simulink library "WECSim_Lib_PTOSim"  (R2020b)
settings: Solver=ode45  StartTime=0.0  StopTime=10.0  RelTol=1e-3  EnableMultiTasking=on
undefined symbols (not defined in the file or in its folder): DiscIntNeverNeededParam, magnitude, ptoSim, simu
libraries: $bdroot x3, simulink x2
(part 1 of 2)
settings Model: RequirementInfo="{}  %GIDa_42666abb_d6d9_408c_ae24_f6520282b61c"  Creator=sor  LastModifiedBy=akeeste
settings DataIOCC: LimitDataPoints=on  SaveFormat=Array  ReturnWorkspaceOutputs=off
settings OptimizationCC: LifeSpan=inf
settings DebuggingCC: SolverPrmCheckMsg=warning  AllowSymbolicDim=off  SFUnexpectedBacktrackingDiag=warning  SFNoUnconditionalDefaultTransitionDiag=warning  SFExecutionAtInitializationDiag=none  ArithmeticOperatorsInVariantConditions=warning
settings HardwareCC: ProdBitPerPointer=32  ProdBitPerSizeT=32  ProdBitPerPtrDiffT=32  ProdLargestAtomicFloat=None  ProdIntDivRoundTo=Undefined  ProdEndianess=Unspecified  ProdWordSize=32  ProdHWDeviceType=32-bit Generic
settings ModelReferenceCC: PropagateSignalLabelsOutOfModel=off
settings SFSimCC: SimUseLocalCustomCode=off  CustomCodeUndefinedFunction=UseInterfaceOnly
settings RTWCC: RTWUseLocalCustomCode=off
settings CodeAppCC: StateflowObjectComments=on
settings GRTTargetCC: TargetLangStandard=C89/C90 (ANSI)
settings ConfigComp: CovMetricSettings=dw  CovSaveCumulativeToWorkspaceVar=on  CovSaveSingleToWorkspaceVar=on  CovExternalEMLEnable=off  CovSFcnEnable=off

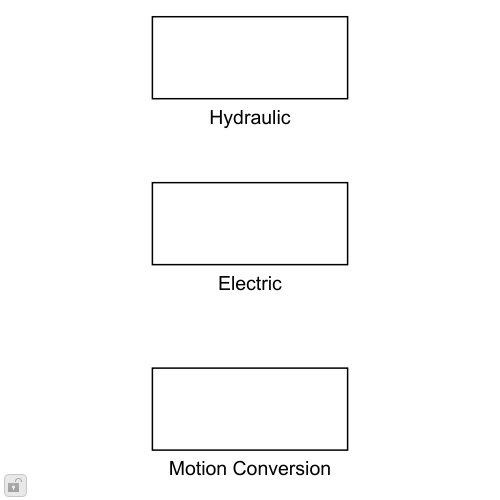
[thumbnail: Simulink's stored preview of the top-level diagram]
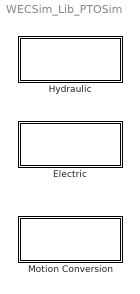
== system WECSim_Lib_PTOSim ==
  Electric : Subsystem  RequirementInfo="{}  %GIDa_5439fdb4_7c29_433c_8677_23bf92e18f11"
  Hydraulic : Subsystem  RequirementInfo={} %GIDa_f12a42eb_b9cb_4818_b573_b7dee4183a3b
  Motion Conversion : Subsystem

== system WECSim_Lib_PTOSim/Electric ==
  Direct Drive Linear Generator : Subsystem  mask{ptoSim=ptoSim(1), InputFiletext=Use WEC-Sim input file to define Direct Drive Linear Generator parameters, Rs=0, Ls=0, Rload=0, Bfric=0, tau_p=0, theta_d_0=0, lambda_sd_0=0, lambda_sq_0=0, lambda_fd=0}
      mask prompts: ptoSim "Direct Drive Linear Generator Name"; Rs "Winding resistance [ohm]"; Ls "Winding inductance [H]"; Rload "External load resistance [ohm]"; Bfric "Friction coefficient [kg/s]"; tau_p "Magnet pole pitch [m]"; theta_d_0 "Initial rotor frame angle [rad]"; lambda_sd_0 "Initial stator d-axis flow linkage"; lambda_sq_0 "Initial stator q-axis flow linkage"; lambda_fd "Flow linkage fd"
      mask init:
      | if exist('ptoSim','var')
      |     h=[gcb '/To Workspace'];
      |     responseName=['ptoSim' num2str(ptoSim.number) '_out'];
      |     set_param(h,'VariableName',responseName);
      | end
      | clear h responseName
      mask DialogControl CustomParameterGroup Prompt: Custom Parameters
      mask DialogControl LGParameters Prompt: Linear Generator Parameters
      mask Display: image('DirectDriveLinearGenerator.png'); % Use "Edit Image" on toolstrip to change.
  Direct Drive Rotary Generator : Subsystem  mask{ptoSim=ptoSim(1)}
      mask prompts: ptoSim "Direct Drive Rotary Generator Name"
      mask init:
      | if exist('ptoSim','var')
      |     h=[gcb '/To Workspace'];
      |     responseName=['ptoSim' num2str(ptoSim.number) '_out'];
      |     set_param(h,'VariableName',responseName);
      | end
      | clear h responseName
      mask Display: image('DirectDriveRotaryGenerator.png'); % Use "Edit Image" on toolstrip to change.
  Electric Generator Equivalent Circuit : Subsystem  mask{ptoSim=ptoSim(1), InputFiletext=Use WEC-Sim input file to define Electric Machine parameters, Ra=0, La=0, Ke=0, bShaft=0, Jem=0}
      mask prompts: ptoSim "Electric Machine Name"; Ra "Armature Resistance [ohm]"; La "Armature Inductance [H]"; Ke "Back-emf or Torque constant [V/(rad/s)]"; bShaft "Rotor Damping [N s/m]"; Jem "Rotor Inertia [kg m^2]"
      mask init:
      | if exist('ptoSim','var')
      |     h=[gcb '/To Workspace'];
      |     responseName=['ptoSim' num2str(ptoSim.number) '_out'];
      |     set_param(h,'VariableName',responseName);
      | end
      | clear h responseName
      settings: PortSchema="{\"entries\":[{\"content\":{\"sides\":[{\"content\":{\"connectorIds\":[\"In1\"]},\"type\":\"ConnectorPlacement.EquallySpacedRectSide\",\"uuid\":\"38b15b7d-d952-45b6-9eb0-5d473736364e\"},{\"content\":{\"connectorIds\":[\"Out1\"],\"side\":\"RIGHT\"},\"type\":\"ConnectorPlacement.EquallySpacedRectSide\",\"uuid\":\"de64adb9-f2de-4dd5-b519-c63af884483d\"},{\"content\":{\"connectorIds\":[\"In2\"],\"side\":\"TOP\"},\"type\":\"ConnectorPlacement.EquallySpacedRectSide\",\"uuid\":\"eaa9506a-5e37-41b4-975c-a8d526700d36\"},{\"content\":{\"connectorIds\":[],\"side\":\"HIDDEN\"},\"type\":\"ConnectorPlacement.EquallySpacedRectSide\",\"uuid\":\"f8da1221-e5bc-4844-b966-beaaa1d6bf60\"}]},\"type\":\"ConnectorPlacement.EquallySpacedConnector\",\"uuid\":\"4da2b473-e94d-42dc-9143-64fbcbf5d9e1\"}],\"packageUris\":[\"http://schema.mathworks.com/mf0/Connector/R2020b\"],\"version\":\"1.0\"}"
      mask DialogControl CustomParameterGroup Prompt: Custom Parameters
      mask DialogControl EMParameters Prompt: Electric Machine Parameters
      mask Display: image('ElectricMotor.png'); % Use "Edit Image" on toolstrip to change.
  Simple Direct Drive PTO : Subsystem  mask{ptoSim=ptoSim(1)}
      mask prompts: ptoSim "Simple Direct Drive PTO"
      mask init:
      | if exist('ptoSim', 'var')
      |     h=[gcb '/To Workspace'];
      |     responseName=['ptoSim' num2str(ptoSim.number) '_out'];
      |     set_param(h,'VariableName',responseName);
      | end
      | clear h responseName
      mask Display: image('simpleDDPTO.png'); % Use "Edit Image" on toolstrip to change.

== system WECSim_Lib_PTOSim/Hydraulic ==
  Check Valve : Subsystem  mask{ptoSim=ptoSim(1)}
      mask prompts: ptoSim "Chack Valve Name"
      mask init:
      | if exist('ptoSim','var')
      |     h=[gcb '/To Workspace'];
      |     responseName=['ptoSim' num2str(ptoSim.number) '_out'];
      |     set_param(h,'VariableName',responseName);
      | end
      | clear h responseName
      mask Display: image('CheckValve.png'); % Use "Edit Image" on toolstrip to change.
  Compressible Fluid Piston : Subsystem  mask{ptoSim=ptoSim(1)}
      mask prompts: ptoSim "Piston Name"
      mask help:
      | PTO-Sim Compressible Fluid Piston
      |
      | This block simualtes a hydraulic cylinder using a compressible fluid model. The block inputs are Response, QA and QB. Response is the signal output of the block Rotational PTO Actuation Force. QA and QB are the flow rate for port A and port B of the cylinder. The outputs of the block are ForcePTO, PA, and PB.
      mask init:
      | if exist('ptoSim','var')
      |     h=[gcb '/To Workspace'];
      |     responseName=['ptoSim' num2str(ptoSim.number) '_out'];
      |     set_param(h,'VariableName',responseName);
      | end
      | clear h responseName
      settings: PortSchema="{\"entries\":[{\"content\":{\"sides\":[{\"content\":{\"connectorIds\":[\"In1\",\"In2\"]},\"type\":\"ConnectorPlacement.EquallySpacedRectSide\",\"uuid\":\"572dbc7c-8f4c-46fc-9000-663c89355fbd\"},{\"content\":{\"connectorIds\":[\"Out1\",\"Out2\",\"Out3\"],\"side\":\"RIGHT\"},\"type\":\"ConnectorPlacement.EquallySpacedRectSide\",\"uuid\":\"3b7821ce-a540-4de1-8f34-0d55375c774c\"},{\"content\":{\"connectorIds\":[\"In3\"],\"side\":\"TOP\"},\"type\":\"ConnectorPlacement.EquallySpacedRectSide\",\"uuid\":\"b6f5c275-868d-447d-b609-cdda14e9f222\"},{\"content\":{\"connectorIds\":[],\"side\":\"HIDDEN\"},\"type\":\"ConnectorPlacement.EquallySpacedRectSide\",\"uuid\":\"5b34aa5d-01fb-4d75-9f22-3e4ce64ee132\"}]},\"type\":\"ConnectorPlacement.EquallySpacedConnector\",\"uuid\":\"5b16a2f7-6624-4a26-89bf-8d87cef610e1\"}],\"packageUris\":[\"http://schema.mathworks.com/mf0/Connector/R2020b\"],\"version\":\"1.0\"}"
      mask Help:
      | This block simualtes a hydraulic cylinder using a compressible fluid model. The block inputs are Response and HydraulicInput. Response is the signal output of the block Rotational PTO Actuation Force. HydraulicInput is a two signal vector with the information of the flow rate for port A and port B of the cylinder. The output of the block is ptoSimOutput, which is a three signal vector with pressureA, pressureB, and forcePTO.
      | 
      | The outputs are calculated using the model presented in the following link: http://wec-sim.github.io/WEC-Sim/master/user/advanced_features.html#pto-sim
      mask Display: image('DoubleActingPiston.png'); % Use "Edit Image" on toolstrip to change.
  Gas-Charged Hydraulic Accumulator : Subsystem  mask{ptoSim=ptoSim(1)}
      mask prompts: ptoSim "Accumulator Name"
      mask init:
      | if exist('ptoSim','var')
      |     h=[gcb '/To Workspace'];
      |     responseName=['ptoSim' num2str(ptoSim.number) '_out'];
      |     set_param(h,'VariableName',responseName);
      | end
      | clear h responseName
      mask Display: image('GasAccumulator.png'); % Use "Edit Image" on toolstrip to change.
  Hydraulic Motor : Subsystem  Variant=on  AllowZeroVariantControls=on  mask{ptoSim=ptoSim(1)}
      mask prompts: ptoSim "Hydraulic Motor Name"
      mask init:
      | if exist('ptoSim','var')
      |     %%
      |     % Analytical efficiency
      |     %%
      |     h = [gcb '/AnalyticalEfficiencyModel'];
      |     responseName = ['sv_b' num2str(ptoSim.number) '_AnalyticalEfficiency'];
      |     set_param(h,'VariantControl',responseName);
      |     %%
      |     % Tabulated Efficiency
      |     %%
      |     h = [gcb '/TabulatedEfficiency'];
      |     responseName = ['sv_b' num2str(ptoSim.number) '_TabulatedEfficiency'];
      |     set_param(h,'VariantControl',responseName);
      |     %%
      |     % Set zero active variant controls to prevent label issue (works 2017b+)
      |     %%
      |     set_param(gcb,'AllowZeroVariantControls','on');
      |     %%
      |     h=[gcb '/TabulatedEfficiency/To Workspace'];
      |     responseName=['ptoSim' num2str(ptoSim.number) '_out'];
      |     set_param(h,'VariableName',responseName);
      |     %%
      |     h=[gcb '/AnalyticalEfficiencyModel/To Workspace'];
      |     responseName=['ptoSim' num2str(ptoSim.number) '_out'];
      |     set_param(h,'VariableName',responseName);
      | end
      | clear h responseName
      mask Display: image('VariableDisplacementHydraulicMotor.png'); % Use "Edit Image" on toolstrip to change.
  Rectifying Check Valve : Subsystem  mask{ptoSim=ptoSim(1)}
      mask prompts: ptoSim "Rectifying Valve Name"
      mask init:
      | if exist('ptoSim','var')
      |     h=[gcb '/To Workspace'];
      |     responseName=['ptoSim' num2str(ptoSim.number) '_out'];
      |     set_param(h,'VariableName',responseName);
      | end
      | clear h responseName
      mask Display: image('RectifyingCheckValve.png'); % Use "Edit Image" on toolstrip to change.

== system WECSim_Lib_PTOSim/Motion Conversion ==
  Rotary to Linear Adjustable Rod : Subsystem  mask{ptoSim=ptoSim(1)}
      mask prompts: ptoSim "Adjustable Rod Name"
      mask init:
      | if exist('ptoSim','var')
      |     h=[gcb '/To Workspace'];
      |     responseName=['ptoSim' num2str(ptoSim.number) '_out'];
      |     set_param(h,'VariableName',responseName);
      | end
      | clear h responseName
  Rotary to Linear Crank : Subsystem  mask{ptoSim=ptoSim(1)}
      mask prompts: ptoSim "Linear Crank Name"
      mask init:
      | if exist('ptoSim','var')
      |     h=[gcb '/To Workspace'];
      |     responseName=['ptoSim' num2str(ptoSim.number) '_out'];
      |     set_param(h,'VariableName',responseName);
      | end
      | clear h responseName

== system WECSim_Lib_PTOSim/Electric/Direct Drive Linear Generator ==
  Response : Inport
  ABCtoDQ : Subsystem
  ABCtoDQ2 : Subsystem
  Add : Sum
  Bus Creator : BusCreator  Inputs=11
  Bus Selector : BusSelector  OutputSignals=velocity
  Demux : Demux  Outputs=3
  Demux1 : Demux  Outputs=3
  Gain : Gain  Gain=-1
  Gain5 : Gain  Gain=2*pi/(2*ptoSim.directLinearGenerator.tau_p)
  Integrator2 : Integrator  InitialCondition=ptoSim.directLinearGenerator.theta_d_0
  Losses : Subsystem
  Product : Product
  Selector1 : Selector  InputPortWidth=6  IndexOptions=Index vector (dialog)  Indices=3  OutputSizes=1
  Subsystem : Subsystem
  Subsystem1 : Subsystem
  Terminator : Terminator
  To Workspace : ToWorkspace  VariableName=ptoSim1_out  SaveFormat=Structure With Time  SampleTime=simu.dtOut
  Force : Outport
  wires:
  Bus Selector/1 -> Selector1/1  "<velocity>"
  Response/1 -> Bus Selector/1
  Gain5/1 -> Subsystem/2(wd), Integrator2/1  "wsyn"
  Selector1/1 -> Bus Creator/10, Product/1, Losses/1(vel), Gain5/1  "vel"
  Integrator2/1 -> ABCtoDQ/1(theta_d), ABCtoDQ2/1(theta_d)
  ABCtoDQ/1(DQ) -> Subsystem/1(vsdq)
  Losses/1(fricForce) -> Add/1, Bus Creator/3  "fricForce"
  Subsystem/1(Fem) -> Add/2
  Subsystem/2(isdq) -> ABCtoDQ2/2(dq)
  ABCtoDQ2/1(abc) -> Demux/1, Subsystem1/1(Iabc)
  Subsystem1/1(Vabc) -> Demux1/1, ABCtoDQ/2(ABC)
  Add/1 -> Product/2, Force/1, Bus Creator/2  "force"
  Product/1 -> Gain/1
  Gain/1 -> Terminator/1, Bus Creator/1  "absPower"
  Bus Creator/1 -> To Workspace/1
  Demux/1 -> Bus Creator/4  "Ia"
  Demux/2 -> Bus Creator/5  "Ib"
  Demux/3 -> Bus Creator/6  "Ic"
  Demux1/3 -> Bus Creator/9  "Vc"
  Demux1/2 -> Bus Creator/8  "Vb"
  Demux1/1 -> Bus Creator/7  "Va"
  Subsystem1/2(elecPower) -> Bus Creator/11  "elecPower"

== system WECSim_Lib_PTOSim/Electric/Direct Drive Rotary Generator ==
  Response : Inport
  ABCtoDQ : Subsystem  AncestorBlock=PTOSim_Lib/Electric/Direct Drive Linear Generator/ABCtoDQ
  ABCtoDQ2 : Subsystem  AncestorBlock=PTOSim_Lib/Electric/Direct Drive Linear Generator/ABCtoDQ2
  Add : Sum
  Bus Creator : BusCreator  Inputs=11
  Bus Selector : BusSelector  OutputSignals=velocity
  Demux : Demux  Outputs=3
  Demux1 : Demux  Outputs=3
  Gain : Gain  Gain=-1
  Gain5 : Gain  Gain=2*pi*ptoSim.directRotaryGenerator.radius/(2*ptoSim.directRotaryGenerator.tau_p)
  Integrator2 : Integrator  InitialCondition=ptoSim.directRotaryGenerator.theta_d_0
  Losses : Subsystem  AncestorBlock=PTOSim_Lib/Electric/Direct Drive Linear Generator/Losses
  Product : Product
  Selector1 : Selector  InputPortWidth=6  IndexOptions=Index vector (dialog)  Indices=3  OutputSizes=1
  Subsystem : Subsystem  AncestorBlock=PTOSim_Lib/Electric/Direct Drive Linear Generator/Subsystem
  Subsystem1 : Subsystem  AncestorBlock=PTOSim_Lib/Electric/Direct Drive Linear Generator/Subsystem1
  Terminator : Terminator
  To Workspace : ToWorkspace  VariableName=ptoSim1_out  SaveFormat=Structure With Time  SampleTime=simu.dtOut
  Torque : Outport
  wires:
  Demux1/2 -> Bus Creator/8  "Vb"
  Selector1/1 -> Bus Creator/10, Product/1, Losses/1(vel), Gain5/1  "vel"
  Subsystem/1(Fem) -> Add/2
  Integrator2/1 -> ABCtoDQ/1(theta_d), ABCtoDQ2/1(theta_d)
  Subsystem/2(isdq) -> ABCtoDQ2/2(dq)
  Gain5/1 -> Subsystem/2(wd), Integrator2/1  "wsyn"
  Subsystem1/1(Vabc) -> Demux1/1, ABCtoDQ/2(ABC)
  Bus Creator/1 -> To Workspace/1
  Demux/3 -> Bus Creator/6  "Ic"
  Add/1 -> Product/2, Torque/1, Bus Creator/2  "Torque"
  Bus Selector/1 -> Selector1/1  "<velocity>"
  Losses/1(fricTorque) -> Add/1, Bus Creator/3  "fricTorque"
  Demux/1 -> Bus Creator/4  "Ia"
  Gain/1 -> Terminator/1, Bus Creator/1  "absPower"
  Demux1/3 -> Bus Creator/9  "Vc"
  Product/1 -> Gain/1
  Response/1 -> Bus Selector/1
  ABCtoDQ2/1(abc) -> Demux/1, Subsystem1/1(Iabc)
  Demux1/1 -> Bus Creator/7  "Va"
  Subsystem1/2(elecPower) -> Bus Creator/11  "elecPower"
  Demux/2 -> Bus Creator/5  "Ib"
  ABCtoDQ/1(DQ) -> Subsystem/1(vsdq)

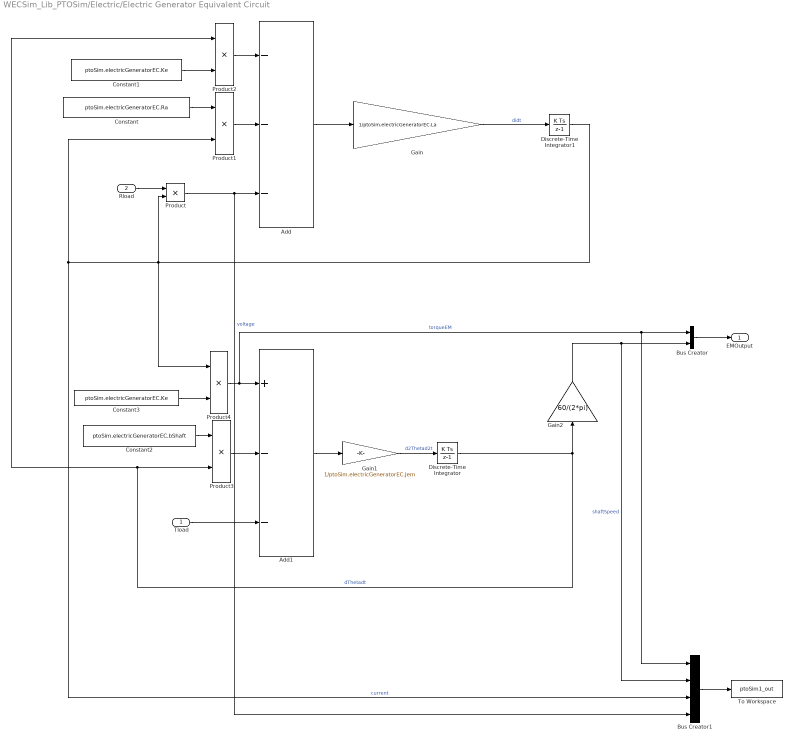
== system WECSim_Lib_PTOSim/Electric/Electric Generator Equivalent Circuit ==
  Tload : Inport
  Rload : Inport  Port=2
  Add : Sum  Inputs=---
  Add1 : Sum  Inputs=+--
  Bus Creator : BusCreator  Inputs=2
  Bus Creator1 : BusCreator  Inputs=4
  Constant : Constant  Value=ptoSim.electricGeneratorEC.Ra
  Constant1 : Constant  Value=ptoSim.electricGeneratorEC.Ke
  Constant2 : Constant  Value=ptoSim.electricGeneratorEC.bShaft
  Constant3 : Constant  Value=ptoSim.electricGeneratorEC.Ke
  Discrete-Time Integrator : DiscreteIntegrator  InitialCondition=(2*pi/60)*ptoSim.electricGeneratorEC.wShaftIni  SampleTime=-1  ICPrevOutput=DiscIntNeverNeededParam  ICPrevScaledInput=DiscIntNeverNeededParam
  Discrete-Time Integrator1 : DiscreteIntegrator  InitialCondition=ptoSim.electricGeneratorEC.currentIni  SampleTime=-1  ICPrevOutput=DiscIntNeverNeededParam  ICPrevScaledInput=DiscIntNeverNeededParam
  Gain : Gain  Gain=1/ptoSim.electricGeneratorEC.La
  Gain1 : Gain  Gain=1/ptoSim.electricGeneratorEC.Jem
  Gain2 : Gain  Gain=60/(2*pi)
  Product{,1..4} (5 alike) : Product
  To Workspace : ToWorkspace  VariableName=ptoSim1_out  SaveFormat=Structure With Time  SampleTime=simu.dtOut
  EMOutput : Outport
  wires:
  Add/1 -> Gain/1
  Gain/1 -> Discrete-Time Integrator1/1  "didt"
  Rload/1 -> Product/1
  Discrete-Time Integrator1/1 -> Product4/1, Product/2, Bus Creator1/3, Product1/2  "current"
  Product/1 -> Bus Creator1/4, Add/3  "voltage"
  Product1/1 -> Add/2
  Constant/1 -> Product1/1
  Product2/1 -> Add/1
  Constant1/1 -> Product2/2
  Tload/1 -> Add1/3
  Add1/1 -> Gain1/1
  Gain1/1 -> Discrete-Time Integrator/1  "d2Thetad2t"
  Product3/1 -> Add1/2
  Constant2/1 -> Product3/1
  Discrete-Time Integrator/1 -> Product2/1, Product3/2, Gain2/1  "dThetadt"
  Product4/1 -> Bus Creator1/1, Bus Creator/1, Add1/1  "torqueEM"
  Constant3/1 -> Product4/2
  Bus Creator/1 -> EMOutput/1
  Gain2/1 -> Bus Creator1/2, Bus Creator/2  "shaftSpeed"
  Bus Creator1/1 -> To Workspace/1

== system WECSim_Lib_PTOSim/Electric/Simple Direct Drive PTO ==
  Control Force : Inport
  Velocity : Inport  Port=2
  Add : Sum  Inputs=+++
  Add1 : Sum
  Bus Creator : BusCreator  Inputs=10
  Control Current Time Constant : TransferFcn  Denominator=[ptoSim.simpleDirectDrivePTO.windingInductance/ptoSim.simpleDirectDrivePTO.windingResistance 1]
  Derivative : Derivative  CoefficientInTFapproximation=1000*2*pi
  Gain : Gain  Gain=-ptoSim.simpleDirectDrivePTO.drivetrainInertia
  Gain1 : Gain  Gain=ptoSim.simpleDirectDrivePTO.torqueConstant
  Gain2 : Gain  Gain=-ptoSim.simpleDirectDrivePTO.drivetrainFriction
  Gain3 : Gain  Gain=ptoSim(1).simpleDirectDrivePTO.windingResistance
  Gain4 : Gain  Gain=1/ptoSim.simpleDirectDrivePTO.torqueConstant
  Magnitude Squared : Math  Operator=magnitude^2  SaturateOnIntegerOverflow=on
  Product : Product
  Product5 : Product
  To Workspace : ToWorkspace  VariableName=ptoSim1_out  SaveFormat=Structure With Time  SampleTime=simu.dtOut
  gear_ratio : Gain  Gain=ptoSim.simpleDirectDrivePTO.gearRatio
  gear_ratio1 : Gain  Gain=1/ptoSim.simpleDirectDrivePTO.gearRatio
  gear_ratio2 : Gain  Gain=ptoSim.simpleDirectDrivePTO.gearRatio
  Force : Outport
  wires:
  Derivative/1 -> Gain/1
  Control Force/1 -> gear_ratio1/1
  Gain/1 -> Bus Creator/4, Add/1  "inertiaForce"
  Control Current Time Constant/1 -> Gain4/1, Add/3, Bus Creator/6  "genForce"
  Velocity/1 -> gear_ratio/1
  Magnitude Squared/1 -> Gain3/1
  Product/1 -> Add1/1
  Gain1/1 -> Product/1, Bus Creator/8  "voltage"
  Gain2/1 -> Add/2, Bus Creator/5  "fricForce"
  Bus Creator/1 -> To Workspace/1
  Gain4/1 -> Magnitude Squared/1, Product/2, Bus Creator/7  "current"
  Product5/1 -> Bus Creator/2  "absPower"
  Gain3/1 -> Add1/2, Bus Creator/9  "I2RLosses"
  Add/1 -> gear_ratio2/1, Bus Creator/3, Product5/2  "force"
  Add1/1 -> Bus Creator/10  "elecPower"
  gear_ratio/1 -> Bus Creator/1, Gain1/1, Gain2/1, Derivative/1, Product5/1  "velocity"
  gear_ratio1/1 -> Control Current Time Constant/1
  gear_ratio2/1 -> Force/1

== system WECSim_Lib_PTOSim/Hydraulic/Check Valve ==
  DeltaP : Inport
  Bus Creator : BusCreator  Inputs=2
  Constant : Constant  Value=ptoSim.checkValve.rho
  Divide : Product  Inputs=/*
  Gain : Gain  Gain=ptoSim.checkValve.k1
  Gain1 : Gain  Gain=2
  Gain2 : Gain  Gain=ptoSim.checkValve.Cd
  Product : Product
  Product1 : Product
  Sqrt : Sqrt  SaturateOnIntegerOverflow=on
  Subsystem : Subsystem
  To Workspace : ToWorkspace  VariableName=ptoSim1_out  SaveFormat=Structure With Time  SampleTime=-1
  Trigonometric Function : Trigonometry  Operator=tanh
  Qcv : Outport
  wires:
  Product1/1 -> Bus Creator/1, Qcv/1  "flowCheckValve"
  DeltaP/1 -> Bus Creator/2, Subsystem/1(DeltaP), Gain/1, Gain1/1  "deltaPCheckValve"
  Subsystem/1(Av) -> Product1/2
  Gain/1 -> Trigonometric Function/1
  Trigonometric Function/1 -> Product/1
  Gain1/1 -> Product/2
  Sqrt/1 -> Gain2/1
  Divide/1 -> Sqrt/1
  Gain2/1 -> Product1/1
  Constant/1 -> Divide/1
  Product/1 -> Divide/2
  Bus Creator/1 -> To Workspace/1

== system WECSim_Lib_PTOSim/Hydraulic/Compressible Fluid Piston ==
  QA : Inport
  QB : Inport  Port=2
  Response : Inport  Port=3
  Add : Sum  Inputs=-+
  Bus Creator1 : BusCreator  Inputs=3
  Bus Selector : BusSelector  OutputSignals=position,velocity
  Constant : Constant  Value=ptoSim.hydPistonCompressible.Ap_B
  Constant1 : Constant  Value=ptoSim.hydPistonCompressible.Ap_A
  Discrete-Time Integrator : DiscreteIntegrator  InitialCondition=ptoSim.hydPistonCompressible.pAi  SampleTime=-1  ICPrevOutput=DiscIntNeverNeededParam  ICPrevScaledInput=DiscIntNeverNeededParam
  Discrete-Time Integrator1 : DiscreteIntegrator  InitialCondition=ptoSim.hydPistonCompressible.pBi  SampleTime=-1  ICPrevOutput=DiscIntNeverNeededParam  ICPrevScaledInput=DiscIntNeverNeededParam
  Product1 : Product
  Product2 : Product
  Selector : Selector  InputPortWidth=6  IndexOptions=Index vector (dialog)  Indices=3  OutputSizes=1
  Selector1 : Selector  InputPortWidth=6  IndexOptions=Index vector (dialog)  Indices=3  OutputSizes=1
  Subsystem : Subsystem  AncestorBlock=PTOSim_Lib_UpdatedV3/Hydraulic/Compressible Fluid Piston Updated/Subsystem
  To Workspace : ToWorkspace  VariableName=ptoSim1_out  SaveFormat=Structure With Time  SampleTime=simu.dtOut
  dPa_dt : Subsystem  AncestorBlock=PTOSim_Lib_UpdatedV3/Hydraulic/Compressible Fluid Piston Updated/dPa_dt
  ForcePTO : Outport
  PA : Outport  Port=2
  PB : Outport  Port=3
  wires:
  QA/1 -> dPa_dt/3(QA)
  Constant1/1 -> Product2/2
  Discrete-Time Integrator1/1 -> Bus Creator1/3, PB/1, Product1/2  "pressureB"
  Selector/1 -> Subsystem/1(Pos), dPa_dt/1(Pos)
  Add/1 -> Bus Creator1/2, ForcePTO/1  "forcePTO"
  Bus Creator1/1 -> To Workspace/1
  QB/1 -> Subsystem/3(QB)
  Product1/1 -> Add/2
  dPa_dt/1(dPA_dt) -> Discrete-Time Integrator/1
  Product2/1 -> Add/1
  Constant/1 -> Product1/1
  Bus Selector/2 -> Selector1/1  "<velocity>"
  Subsystem/1(dPB_dt) -> Discrete-Time Integrator1/1
  Selector1/1 -> Subsystem/2(Vel), dPa_dt/2(Vel)
  Response/1 -> Bus Selector/1
  Discrete-Time Integrator/1 -> PA/1, Bus Creator1/1, Product2/1  "pressureA"
  Bus Selector/1 -> Selector/1  "<position>"

== system WECSim_Lib_PTOSim/Hydraulic/Gas-Charged Hydraulic Accumulator ==
  FlowRate : Inport
  Add1 : Sum  Inputs=-+
  Bus Creator : BusCreator  Inputs=2
  Constant4 : Constant  Value=ptoSim.gasHydAccumulator.pIprecharge
  Constant5 : Constant  Value=ptoSim.gasHydAccumulator.vI0
  Constant6 : Constant  Value=ptoSim.gasHydAccumulator.vI0
  Constant7 : Constant  Value=1.4
  Discrete-Time Integrator1 : DiscreteIntegrator  SampleTime=-1  ICPrevOutput=DiscIntNeverNeededParam  ICPrevScaledInput=DiscIntNeverNeededParam
  Divide2 : Product  Inputs=*/
  Math Function1 : Math  Operator=pow  SaturateOnIntegerOverflow=on
  Product : Product
  To Workspace : ToWorkspace  VariableName=ptoSim1_out  SaveFormat=Structure With Time  SampleTime=simu.dtOut
  Pressure : Outport
  wires:
  Constant4/1 -> Product/1
  Constant5/1 -> Divide2/1
  Constant6/1 -> Add1/2
  Discrete-Time Integrator1/1 -> Add1/1
  FlowRate/1 -> Bus Creator/2, Discrete-Time Integrator1/1  "flowRate"
  Add1/1 -> Divide2/2
  Divide2/1 -> Math Function1/1
  Constant7/1 -> Math Function1/2
  Math Function1/1 -> Product/2
  Product/1 -> Bus Creator/1, Pressure/1  "pressure"
  Bus Creator/1 -> To Workspace/1

== system WECSim_Lib_PTOSim/Hydraulic/Hydraulic Motor ==
  note: 1) Add Subsystem or Model blocks as valid variant choices.
      | 2) You cannot connect blocks at this level. At simulation, connectivity is automatically
      | determined, based on the active variant and port name matching.
  Displ : Inport
  DeltaP : Inport  Port=2
  ShaftSpeed : Inport  Port=3
  AnalyticalEfficiencyModel : Subsystem  VariantControl=sv_b1_AnalyticalEfficiency
  TabulatedEfficiency : Subsystem  VariantControl=sv_b1_TabulatedEfficiency
  Torque : Outport
  FlowRate : Outport  Port=2

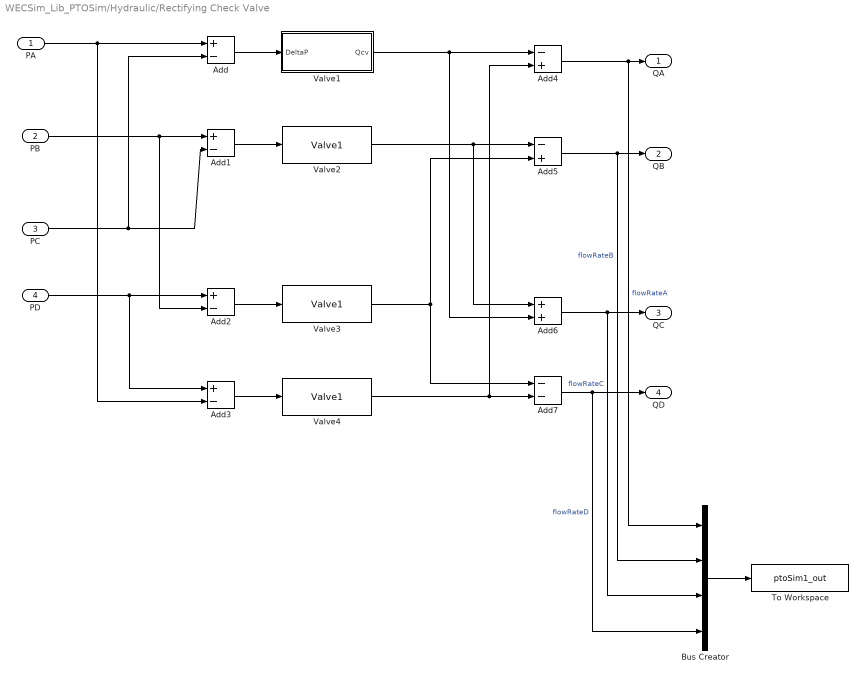
== system WECSim_Lib_PTOSim/Hydraulic/Rectifying Check Valve ==
  PA : Inport
  PB : Inport  Port=2
  PC : Inport  Port=3
  PD : Inport  Port=4
  Add{,1..3} (4 alike) : Sum  Inputs=+-
  Add4 : Sum  Inputs=-+
  Add5 : Sum  Inputs=-+
  Add6 : Sum
  Add7 : Sum  Inputs=--
  Bus Creator : BusCreator  Inputs=4
  To Workspace : ToWorkspace  VariableName=ptoSim1_out  SaveFormat=Structure With Time  SampleTime=-1
  Valve1 : Subsystem
  Valve2 : $bdroot/Hydraulic/Rectifying Check Valve/Valve1  SystemSampleTime=-1  VariantActivationTime=update diagram  Latency=0  AutoFrameSizeCalculation=off
  Valve3 : $bdroot/Hydraulic/Rectifying Check Valve/Valve1  SystemSampleTime=-1  VariantActivationTime=update diagram  Latency=0  AutoFrameSizeCalculation=off
  Valve4 : $bdroot/Hydraulic/Rectifying Check Valve/Valve1  SystemSampleTime=-1  VariantActivationTime=update diagram  Latency=0  AutoFrameSizeCalculation=off
  QA : Outport
  QB : Outport  Port=2
  QC : Outport  Port=3
  QD : Outport  Port=4
  wires:
  Add/1 -> Valve1/1(DeltaP)
  PA/1 -> Add3/2, Add/1
  PC/1 -> Add/2, Add1/2
  Add1/1 -> Valve2/1
  PB/1 -> Add2/2, Add1/1
  Add2/1 -> Valve3/1
  PD/1 -> Add3/1, Add2/1
  Add3/1 -> Valve4/1
  Valve1/1(Qcv) -> Add6/2, Add4/1
  Valve4/1 -> Add7/2, Add4/2
  Valve2/1 -> Add6/1, Add5/1
  Valve3/1 -> Add7/1, Add5/2
  Add7/1 -> Bus Creator/4, QD/1  "flowRateD"
  Add6/1 -> Bus Creator/3, QC/1  "flowRateC"
  Add5/1 -> Bus Creator/2, QB/1  "flowRateB"
  Bus Creator/1 -> To Workspace/1
  Add4/1 -> Bus Creator/1, QA/1  "flowRateA"

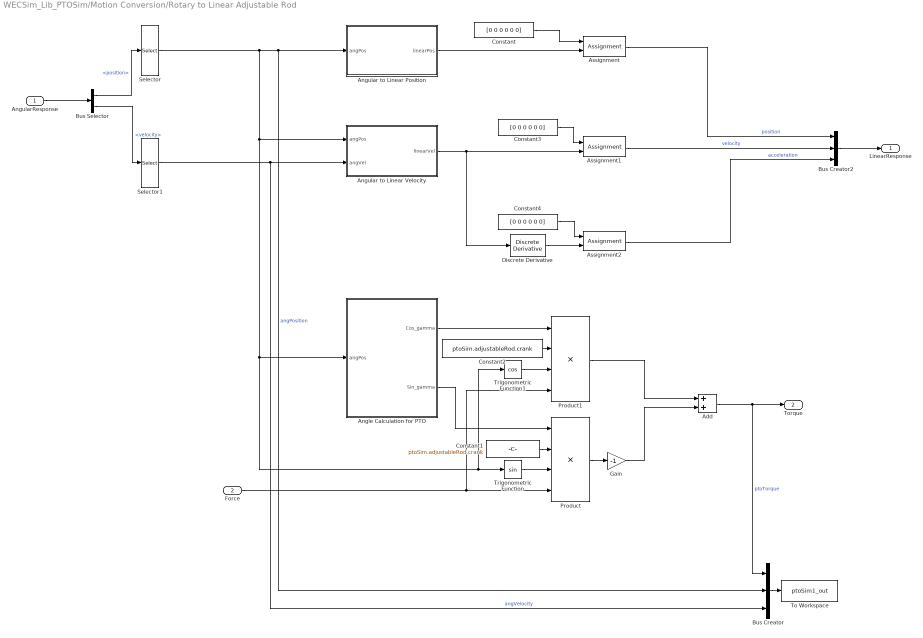
== system WECSim_Lib_PTOSim/Motion Conversion/Rotary to Linear Adjustable Rod ==
  AngularResponse : Inport
  Force : Inport  Port=2
  Add : Sum
  Angle Calculation for PTO : Subsystem
  Angular to Linear Position : Subsystem
  Angular to Linear Velocity : Subsystem
  Assignment : Assignment  IndexOptions=Index vector (dialog)  Indices=3  OutputSizes=1
  Assignment1 : Assignment  IndexOptions=Index vector (dialog)  Indices=3  OutputSizes=1
  Assignment2 : Assignment  IndexOptions=Index vector (dialog)  Indices=3  OutputSizes=1
  Bus Creator : BusCreator  Inputs=3
  Bus Creator2 : BusCreator  Inputs=3
  Bus Selector : BusSelector  OutputSignals=position,velocity
  Constant : Constant  Value=[0 0 0 0 0 0]
  Constant1 : Constant  Value=ptoSim.adjustableRod.crank
  Constant2 : Constant  Value=ptoSim.adjustableRod.crank
  Constant3 : Constant  Value=[0 0 0 0 0 0]
  Constant4 : Constant  Value=[0 0 0 0 0 0]
  Discrete Derivative : simulink/Discrete/Discrete Derivative  gainval=1.0  ICPrevScaledInput=0.0  OutMin=[]  OutMax=[]  OutDataType=fixdt(1, 16)  OutScaling=2^-10  DoSatur=off
  Gain : Gain  Gain=-1
  Product : Product  Inputs=4
  Product1 : Product  Inputs=4
  Selector : Selector  InputPortWidth=6  IndexOptions=Index vector (dialog)  Indices=5  OutputSizes=1
  Selector1 : Selector  InputPortWidth=6  IndexOptions=Index vector (dialog)  Indices=5  OutputSizes=1
  To Workspace : ToWorkspace  VariableName=ptoSim1_out  SaveFormat=Structure With Time  SampleTime=-1
      settings: Decimation=round(simu.dtOut/simu.dt,0)
  Trigonometric Function : Trigonometry
  Trigonometric Function1 : Trigonometry  Operator=cos
  LinearResponse : Outport
  Torque : Outport  Port=2
  wires:
  Angular to Linear Position/1(linearPos) -> Assignment/2
  Selector1/1 -> Bus Creator/3, Angular to Linear Velocity/2(angVel)  "angVelocity"
  Add/1 -> Torque/1, Bus Creator/1  "ptoTorque"
  Bus Creator/1 -> To Workspace/1
  Selector/1 -> Angular to Linear Velocity/1(angPos), Trigonometric Function1/1, Trigonometric Function/1, Angle Calculation for PTO/1(angPos), Bus Creator/2, Angular to Linear Position/1(angPos)  "angPosition"
  Product1/1 -> Add/1
  Gain/1 -> Add/2
  Angle Calculation for PTO/2(Sin_gamma) -> Product/1
  Trigonometric Function1/1 -> Product1/3
  Angle Calculation for PTO/1(Cos_gamma) -> Product1/1
  Force/1 -> Product1/4, Product/4
  Constant2/1 -> Product1/2
  Trigonometric Function/1 -> Product/3
  Constant1/1 -> Product/2
  Product/1 -> Gain/1
  Constant/1 -> Assignment/1
  Constant3/1 -> Assignment1/1
  Angular to Linear Velocity/1(linearVel) -> Discrete Derivative/1, Assignment1/2
  Assignment/1 -> Bus Creator2/1  "position"
  Assignment1/1 -> Bus Creator2/2  "velocity"
  Constant4/1 -> Assignment2/1
  Discrete Derivative/1 -> Assignment2/2
  Assignment2/1 -> Bus Creator2/3  "acceleration"
  Bus Creator2/1 -> LinearResponse/1
  Bus Selector/1 -> Selector/1  "<position>"
  Bus Selector/2 -> Selector1/1  "<velocity>"
  AngularResponse/1 -> Bus Selector/1

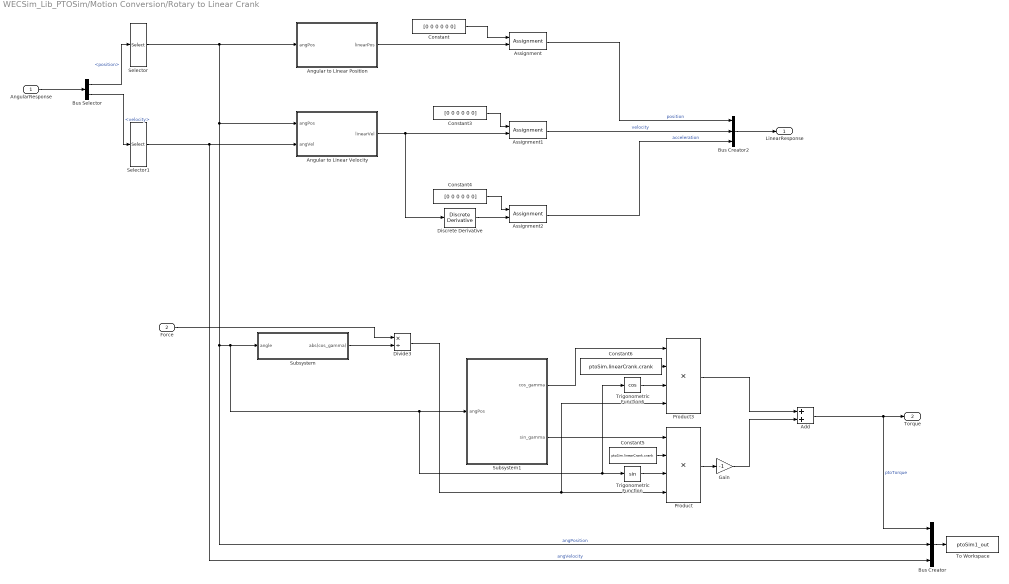
== system WECSim_Lib_PTOSim/Motion Conversion/Rotary to Linear Crank ==
  AngularResponse : Inport
  Force : Inport  Port=2
  Add : Sum
  Angular to Linear Position : Subsystem
  Angular to Linear Velocity : Subsystem
  Assignment : Assignment  IndexOptions=Index vector (dialog)  Indices=3  OutputSizes=1
  Assignment1 : Assignment  IndexOptions=Index vector (dialog)  Indices=3  OutputSizes=1
  Assignment2 : Assignment  IndexOptions=Index vector (dialog)  Indices=3  OutputSizes=1
  Bus Creator : BusCreator  Inputs=3
  Bus Creator2 : BusCreator  Inputs=3
  Bus Selector : BusSelector  OutputSignals=position,velocity
  Constant : Constant  Value=[0 0 0 0 0 0]
  Constant3 : Constant  Value=[0 0 0 0 0 0]
  Constant4 : Constant  Value=[0 0 0 0 0 0]
  Constant5 : Constant  Value=ptoSim.linearCrank.crank
  Constant6 : Constant  Value=ptoSim.linearCrank.crank
  Discrete Derivative : simulink/Discrete/Discrete Derivative  gainval=1.0  ICPrevScaledInput=0.0  OutMin=[]  OutMax=[]  OutDataType=fixdt(1, 16)  OutScaling=2^-10  DoSatur=off
  Divide3 : Product  Inputs=*/
  Gain : Gain  Gain=-1
  Product : Product  Inputs=4
  Product3 : Product  Inputs=4
  Selector : Selector  InputPortWidth=6  IndexOptions=Index vector (dialog)  Indices=5  OutputSizes=1
  Selector1 : Selector  InputPortWidth=6  IndexOptions=Index vector (dialog)  Indices=5  OutputSizes=1
  Subsystem : Subsystem
  Subsystem1 : Subsystem  AncestorBlock=PTOSim_Lib/Motion Conversion/Rotary to Linear Adjustable Rod/Subsystem
  To Workspace : ToWorkspace  VariableName=ptoSim1_out  SaveFormat=Structure With Time  SampleTime=-1
      settings: Decimation=round(simu.dtOut/simu.dt,0)
  Trigonometric Function : Trigonometry
  Trigonometric Function6 : Trigonometry  Operator=cos
  LinearResponse : Outport
  Torque : Outport  Port=2
  wires:
  Selector1/1 -> Bus Creator/3, Angular to Linear Velocity/2(angVel)  "angVelocity"
  Add/1 -> Bus Creator/1, Torque/1  "ptoTorque"
  Bus Creator/1 -> To Workspace/1
  Subsystem/1(abs(cos_gamma)) -> Divide3/2
  Force/1 -> Divide3/1
  Trigonometric Function6/1 -> Product3/3
  Subsystem1/1(cos_gamma) -> Product3/1
  Constant6/1 -> Product3/2
  Divide3/1 -> Product/4, Product3/4
  Gain/1 -> Add/2
  Product3/1 -> Add/1
  Subsystem1/2(sin_gamma) -> Product/1
  Selector/1 -> Angular to Linear Velocity/1(angPos), Subsystem1/1(angPos), Trigonometric Function/1, Trigonometric Function6/1, Subsystem/1(angle), Bus Creator/2, Angular to Linear Position/1(angPos)  "angPosition"
  Trigonometric Function/1 -> Product/3
  Constant5/1 -> Product/2
  Product/1 -> Gain/1
  Bus Selector/2 -> Selector1/1  "<velocity>"
  Bus Selector/1 -> Selector/1  "<position>"
  AngularResponse/1 -> Bus Selector/1
  Constant/1 -> Assignment/1
  Assignment1/1 -> Bus Creator2/2  "velocity"
  Constant4/1 -> Assignment2/1
  Discrete Derivative/1 -> Assignment2/2
  Angular to Linear Velocity/1(linearVel) -> Discrete Derivative/1, Assignment1/2
  Assignment2/1 -> Bus Creator2/3  "acceleration"
  Constant3/1 -> Assignment1/1
  Assignment/1 -> Bus Creator2/1  "position"
  Angular to Linear Position/1(linearPos) -> Assignment/2
  Bus Creator2/1 -> LinearResponse/1

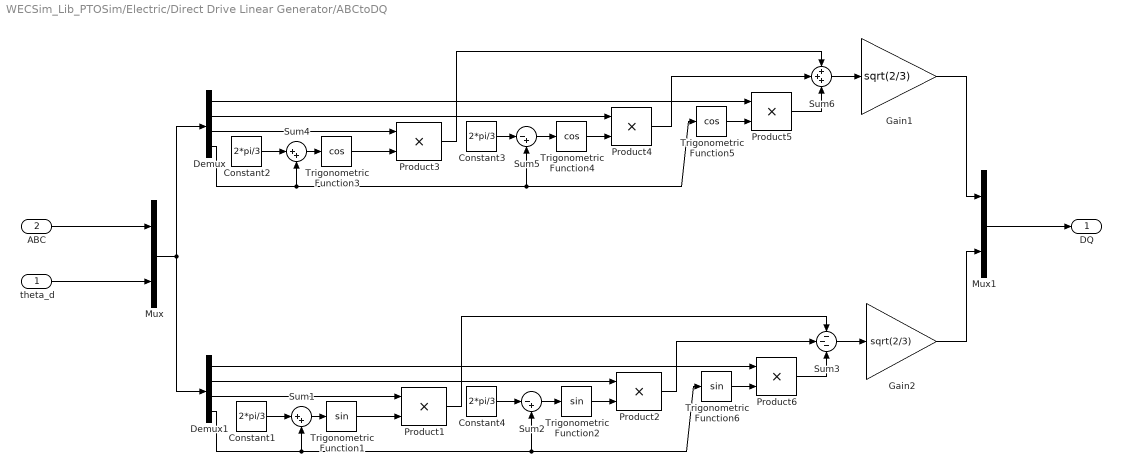
== system WECSim_Lib_PTOSim/Electric/Direct Drive Linear Generator/ABCtoDQ ==
  theta_d : Inport
  ABC : Inport  Port=2
  Constant{1..4} (4 alike) : Constant  Value=2*pi/3
  Demux : Demux
      settings: DisplayOption=none
  Demux1 : Demux
      settings: DisplayOption=none
  Gain1 : Gain  Gain=sqrt(2/3)  SaturateOnIntegerOverflow=on  OutDataTypeStr=Inherit: Same as input  ParamDataTypeStr=Inherit: Same as input
  Gain2 : Gain  Gain=sqrt(2/3)  SaturateOnIntegerOverflow=on  OutDataTypeStr=Inherit: Same as input  ParamDataTypeStr=Inherit: Same as input
  Mux : Mux  Inputs=2
  Mux1 : Mux  Inputs=2
  Product{1..6} (6 alike) : Product  InputSameDT=on  SaturateOnIntegerOverflow=on  OutDataTypeStr=Inherit: Same as first input
  Sum1 : Sum  Inputs=|++  InputSameDT=on  SaturateOnIntegerOverflow=on  OutDataTypeStr=Inherit: Same as first input
  Sum2 : Sum  Inputs=|-+  InputSameDT=on  SaturateOnIntegerOverflow=on  OutDataTypeStr=Inherit: Same as first input
  Sum3 : Sum  Inputs=---  InputSameDT=on  SaturateOnIntegerOverflow=on  OutDataTypeStr=Inherit: Same as first input
  Sum4 : Sum  Inputs=|++  InputSameDT=on  SaturateOnIntegerOverflow=on  OutDataTypeStr=Inherit: Same as first input
  Sum5 : Sum  Inputs=|-+  InputSameDT=on  SaturateOnIntegerOverflow=on  OutDataTypeStr=Inherit: Same as first input
  Sum6 : Sum  Inputs=+++  InputSameDT=on  SaturateOnIntegerOverflow=on  OutDataTypeStr=Inherit: Same as first input
  Trigonometric Function1 : Trigonometry
  Trigonometric Function2 : Trigonometry
  Trigonometric Function3 : Trigonometry  Operator=cos
  Trigonometric Function4 : Trigonometry  Operator=cos
  Trigonometric Function5 : Trigonometry  Operator=cos
  Trigonometric Function6 : Trigonometry
  DQ : Outport
  wires:
  Trigonometric Function4/1 -> Product4/2
  Product5/1 -> Sum6/3
  Demux/1 -> Product5/1
  Product1/1 -> Sum3/1
  Gain1/1 -> Mux1/1
  Sum2/1 -> Trigonometric Function2/1
  Demux1/3 -> Product1/1
  Constant1/1 -> Sum1/1
  Sum1/1 -> Trigonometric Function1/1
  Demux1/1 -> Product6/1
  Demux1/2 -> Product2/1
  Constant4/1 -> Sum2/1
  Sum3/1 -> Gain2/1
  Trigonometric Function1/1 -> Product1/2
  Sum4/1 -> Trigonometric Function3/1
  Product3/1 -> Sum6/1
  Trigonometric Function6/1 -> Product6/2
  Demux1/4 -> Sum1/2, Trigonometric Function6/1, Sum2/2
  Trigonometric Function2/1 -> Product2/2
  Gain2/1 -> Mux1/2
  Demux/4 -> Sum5/2, Trigonometric Function5/1, Sum4/2
  Product2/1 -> Sum3/2
  Mux/1 -> Demux/1, Demux1/1
  Demux/3 -> Product3/1
  Demux/2 -> Product4/1
  Trigonometric Function3/1 -> Product3/2
  Sum6/1 -> Gain1/1
  Trigonometric Function5/1 -> Product5/2
  Product4/1 -> Sum6/2
  Mux1/1 -> DQ/1
  Product6/1 -> Sum3/3
  Constant2/1 -> Sum4/1
  Constant3/1 -> Sum5/1
  Sum5/1 -> Trigonometric Function4/1
  theta_d/1 -> Mux/2
  ABC/1 -> Mux/1

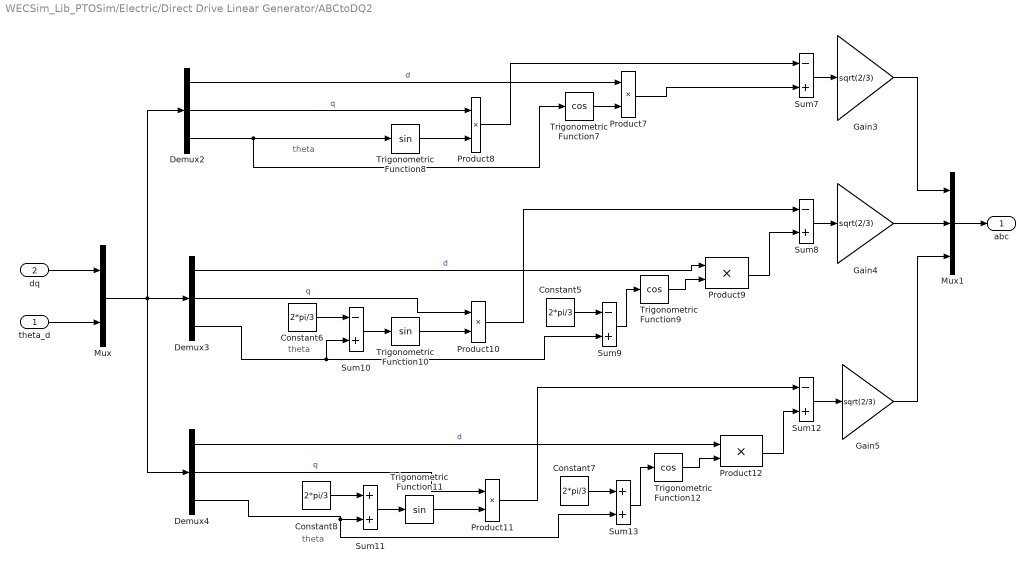
== system WECSim_Lib_PTOSim/Electric/Direct Drive Linear Generator/ABCtoDQ2 ==
  note: theta
  note: theta
  note: theta
  theta_d : Inport
  dq : Inport  Port=2
  Constant{5..8} (4 alike) : Constant  Value=2*pi/3
  Demux2 : Demux  Outputs=3
      settings: DisplayOption=none
  Demux3 : Demux  Outputs=3
      settings: DisplayOption=none
  Demux4 : Demux  Outputs=3
      settings: DisplayOption=none
  Gain3 : Gain  Gain=sqrt(2/3)  SaturateOnIntegerOverflow=on  OutDataTypeStr=Inherit: Same as input  ParamDataTypeStr=Inherit: Same as input
  Gain4 : Gain  Gain=sqrt(2/3)  SaturateOnIntegerOverflow=on  OutDataTypeStr=Inherit: Same as input  ParamDataTypeStr=Inherit: Same as input
  Gain5 : Gain  Gain=sqrt(2/3)  SaturateOnIntegerOverflow=on  OutDataTypeStr=Inherit: Same as input  ParamDataTypeStr=Inherit: Same as input
  Mux : Mux  Inputs=2
  Mux1 : Mux  Inputs=3
  Product{7..12} (6 alike) : Product  InputSameDT=on  SaturateOnIntegerOverflow=on  OutDataTypeStr=Inherit: Same as first input
  Sum{7..10,12} (5 alike) : Sum  Inputs=-+  InputSameDT=on  SaturateOnIntegerOverflow=on  OutDataTypeStr=Inherit: Same as first input
  Sum11 : Sum  InputSameDT=on  SaturateOnIntegerOverflow=on  OutDataTypeStr=Inherit: Same as first input
  Sum13 : Sum  InputSameDT=on  SaturateOnIntegerOverflow=on  OutDataTypeStr=Inherit: Same as first input
  Trigonometric Function10 : Trigonometry
  Trigonometric Function11 : Trigonometry
  Trigonometric Function12 : Trigonometry  Operator=cos
  Trigonometric Function7 : Trigonometry  Operator=cos
  Trigonometric Function8 : Trigonometry
  Trigonometric Function9 : Trigonometry  Operator=cos
  abc : Outport
  wires:
  Trigonometric Function7/1 -> Product7/2
  Constant6/1 -> Sum10/1
  Sum7/1 -> Gain3/1
  Trigonometric Function11/1 -> Product11/2
  Constant5/1 -> Sum9/1
  Product10/1 -> Sum8/1
  Sum11/1 -> Trigonometric Function11/1
  Demux2/3 -> Trigonometric Function8/1, Trigonometric Function7/1
  Demux2/2 -> Product8/1  "q"
  Demux2/1 -> Product7/1  "d"
  Demux3/2 -> Product10/1  "q"
  Product7/1 -> Sum7/2
  Trigonometric Function9/1 -> Product9/2
  Mux/1 -> Demux4/1, Demux2/1, Demux3/1
  Trigonometric Function12/1 -> Product12/2
  Sum13/1 -> Trigonometric Function12/1
  Sum10/1 -> Trigonometric Function10/1
  Trigonometric Function8/1 -> Product8/2
  Gain5/1 -> Mux1/3
  Sum8/1 -> Gain4/1
  Demux3/3 -> Sum10/2, Sum9/2
  Sum9/1 -> Trigonometric Function9/1
  Demux3/1 -> Product9/1  "d"
  Constant7/1 -> Sum13/1
  Demux4/3 -> Sum13/2, Sum11/2
  Product11/1 -> Sum12/1
  Demux4/1 -> Product12/1  "d"
  Demux4/2 -> Product11/1  "q"
  Gain4/1 -> Mux1/2
  Product8/1 -> Sum7/1
  Product9/1 -> Sum8/2
  Gain3/1 -> Mux1/1
  Product12/1 -> Sum12/2
  Constant8/1 -> Sum11/1
  Sum12/1 -> Gain5/1
  Trigonometric Function10/1 -> Product10/2
  Mux1/1 -> abc/1
  theta_d/1 -> Mux/2
  dq/1 -> Mux/1

== system WECSim_Lib_PTOSim/Electric/Direct Drive Linear Generator/Losses ==
  vel : Inport
  Gain : Gain  Gain=ptoSim.directLinearGenerator.Bfric
  fricForce : Outport
  wires:
  vel/1 -> Gain/1
  Gain/1 -> fricForce/1

== system WECSim_Lib_PTOSim/Electric/Direct Drive Linear Generator/Subsystem ==
  vsdq : Inport
  wd : Inport  Port=2
  Add : Sum  Inputs=+-+
  Add1 : Sum  Inputs=--+
  Demux2 : Demux  Outputs=2
      settings: DisplayOption=none
  Fcn : Fcn  Expr=( u(1) - ptoSim.directLinearGenerator.lambda_fd ) / ptoSim.directLinearGenerator.Ls
  Gain : Gain  Gain=1/ptoSim.directLinearGenerator.Ls
  Gain1 : Gain  Gain=pi/ptoSim.directLinearGenerator.tau_p*ptoSim.directLinearGenerator.lambda_fd
  Gain2 : Gain  Gain=ptoSim.directLinearGenerator.Rs
  Gain3 : Gain  Gain=ptoSim.directLinearGenerator.Rs
  Integrator : Integrator  InitialCondition=ptoSim.directLinearGenerator.lambda_sd_0
  Integrator1 : Integrator  InitialCondition=ptoSim.directLinearGenerator.lambda_sq_0
  Mux : Mux  Inputs=2
  Product : Product  RndMeth=Zero
  Product1 : Product  RndMeth=Zero
  Fem : Outport
  isdq : Outport  Port=2
  wires:
  vsdq/1 -> Demux2/1  "vsdq"
  Gain1/1 -> Fem/1
  Mux/1 -> isdq/1  "isdq"
  Gain3/1 -> Add/2  "isd_Rs"
  Add/1 -> Integrator/1  "d_dt_lambda_sd"
  Integrator/1 -> Product1/2, Fcn/1  "lambda_sd"
  Add1/1 -> Integrator1/1  "d_dt_lambda_sq"
  Integrator1/1 -> Gain/1, Product/2  "lambda_sq"
  Demux2/1 -> Add/3  "vsd"
  Product1/1 -> Add1/1
  Demux2/2 -> Add1/3  "vsq"
  Gain2/1 -> Add1/2
  Fcn/1 -> Gain3/1, Mux/1  "isd"
  wd/1 -> Product1/1, Product/1
  Gain/1 -> Gain2/1, Mux/2, Gain1/1  "isq"
  Product/1 -> Add/1

== system WECSim_Lib_PTOSim/Electric/Direct Drive Linear Generator/Subsystem1 ==
  Iabc : Inport
  Gain : Gain  Gain=-1
  Gain1 : Gain  Gain=ptoSim.directLinearGenerator.Rload
  Product : Product
  Sum of Elements : Sum  Inputs=+
  Vabc : Outport
  elecPower : Outport  Port=2
  wires:
  Sum of Elements/1 -> Gain/1
  Iabc/1 -> Gain1/1, Product/2
  Product/1 -> Sum of Elements/1
  Gain/1 -> elecPower/1  "elecPower"
  Gain1/1 -> Vabc/1, Product/1

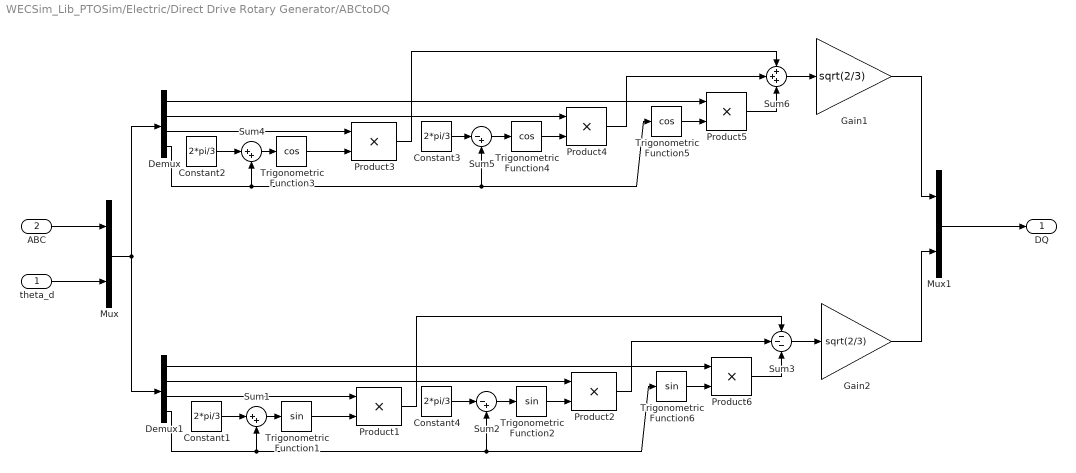
== system WECSim_Lib_PTOSim/Electric/Direct Drive Rotary Generator/ABCtoDQ ==
  theta_d : Inport
  ABC : Inport  Port=2
  Constant{1..4} (4 alike) : Constant  Value=2*pi/3
  Demux : Demux
      settings: DisplayOption=none
  Demux1 : Demux
      settings: DisplayOption=none
  Gain1 : Gain  Gain=sqrt(2/3)  SaturateOnIntegerOverflow=on  OutDataTypeStr=Inherit: Same as input  ParamDataTypeStr=Inherit: Same as input
  Gain2 : Gain  Gain=sqrt(2/3)  SaturateOnIntegerOverflow=on  OutDataTypeStr=Inherit: Same as input  ParamDataTypeStr=Inherit: Same as input
  Mux : Mux  Inputs=2
  Mux1 : Mux  Inputs=2
  Product{1..6} (6 alike) : Product  InputSameDT=on  SaturateOnIntegerOverflow=on  OutDataTypeStr=Inherit: Same as first input
  Sum1 : Sum  Inputs=|++  InputSameDT=on  SaturateOnIntegerOverflow=on  OutDataTypeStr=Inherit: Same as first input
  Sum2 : Sum  Inputs=|-+  InputSameDT=on  SaturateOnIntegerOverflow=on  OutDataTypeStr=Inherit: Same as first input
  Sum3 : Sum  Inputs=---  InputSameDT=on  SaturateOnIntegerOverflow=on  OutDataTypeStr=Inherit: Same as first input
  Sum4 : Sum  Inputs=|++  InputSameDT=on  SaturateOnIntegerOverflow=on  OutDataTypeStr=Inherit: Same as first input
  Sum5 : Sum  Inputs=|-+  InputSameDT=on  SaturateOnIntegerOverflow=on  OutDataTypeStr=Inherit: Same as first input
  Sum6 : Sum  Inputs=+++  InputSameDT=on  SaturateOnIntegerOverflow=on  OutDataTypeStr=Inherit: Same as first input
  Trigonometric Function1 : Trigonometry
  Trigonometric Function2 : Trigonometry
  Trigonometric Function3 : Trigonometry  Operator=cos
  Trigonometric Function4 : Trigonometry  Operator=cos
  Trigonometric Function5 : Trigonometry  Operator=cos
  Trigonometric Function6 : Trigonometry
  DQ : Outport
  wires:
  Trigonometric Function4/1 -> Product4/2
  Product5/1 -> Sum6/3
  Demux/1 -> Product5/1
  Product1/1 -> Sum3/1
  Gain1/1 -> Mux1/1
  Sum2/1 -> Trigonometric Function2/1
  Demux1/3 -> Product1/1
  Constant1/1 -> Sum1/1
  Sum1/1 -> Trigonometric Function1/1
  Demux1/1 -> Product6/1
  Demux1/2 -> Product2/1
  Constant4/1 -> Sum2/1
  Sum3/1 -> Gain2/1
  Trigonometric Function1/1 -> Product1/2
  Sum4/1 -> Trigonometric Function3/1
  Product3/1 -> Sum6/1
  Trigonometric Function6/1 -> Product6/2
  Demux1/4 -> Sum1/2, Trigonometric Function6/1, Sum2/2
  Trigonometric Function2/1 -> Product2/2
  Gain2/1 -> Mux1/2
  Demux/4 -> Sum5/2, Trigonometric Function5/1, Sum4/2
  Product2/1 -> Sum3/2
  Mux/1 -> Demux/1, Demux1/1
  Demux/3 -> Product3/1
  Demux/2 -> Product4/1
  Trigonometric Function3/1 -> Product3/2
  Sum6/1 -> Gain1/1
  Trigonometric Function5/1 -> Product5/2
  Product4/1 -> Sum6/2
  Mux1/1 -> DQ/1
  Product6/1 -> Sum3/3
  Constant2/1 -> Sum4/1
  Constant3/1 -> Sum5/1
  Sum5/1 -> Trigonometric Function4/1
  theta_d/1 -> Mux/2
  ABC/1 -> Mux/1

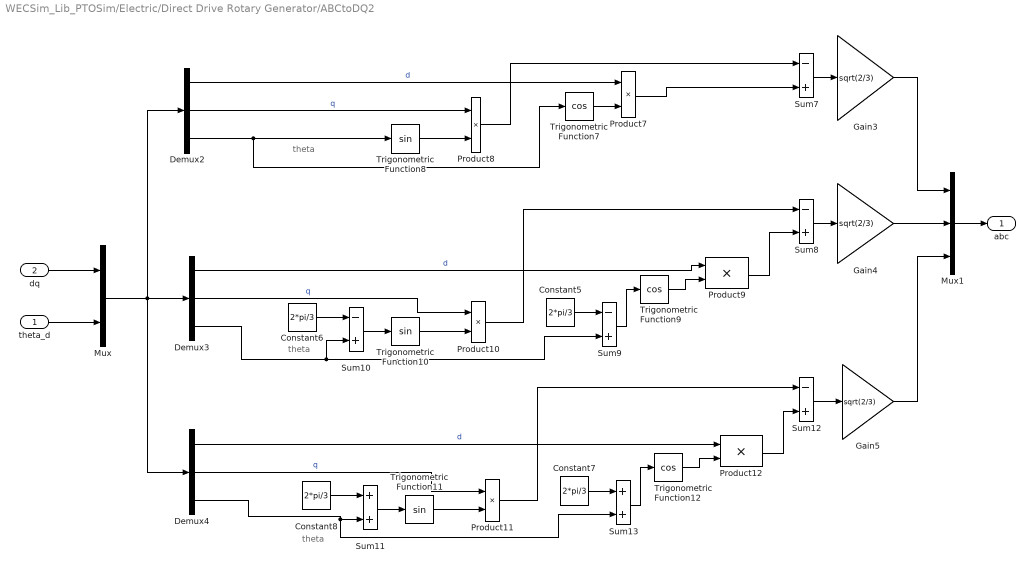
== system WECSim_Lib_PTOSim/Electric/Direct Drive Rotary Generator/ABCtoDQ2 ==
  note: theta
  note: theta
  note: theta
  theta_d : Inport
  dq : Inport  Port=2
  Constant{5..8} (4 alike) : Constant  Value=2*pi/3
  Demux2 : Demux  Outputs=3
      settings: DisplayOption=none
  Demux3 : Demux  Outputs=3
      settings: DisplayOption=none
  Demux4 : Demux  Outputs=3
      settings: DisplayOption=none
  Gain3 : Gain  Gain=sqrt(2/3)  SaturateOnIntegerOverflow=on  OutDataTypeStr=Inherit: Same as input  ParamDataTypeStr=Inherit: Same as input
  Gain4 : Gain  Gain=sqrt(2/3)  SaturateOnIntegerOverflow=on  OutDataTypeStr=Inherit: Same as input  ParamDataTypeStr=Inherit: Same as input
  Gain5 : Gain  Gain=sqrt(2/3)  SaturateOnIntegerOverflow=on  OutDataTypeStr=Inherit: Same as input  ParamDataTypeStr=Inherit: Same as input
  Mux : Mux  Inputs=2
  Mux1 : Mux  Inputs=3
  Product{7..12} (6 alike) : Product  InputSameDT=on  SaturateOnIntegerOverflow=on  OutDataTypeStr=Inherit: Same as first input
  Sum{7..10,12} (5 alike) : Sum  Inputs=-+  InputSameDT=on  SaturateOnIntegerOverflow=on  OutDataTypeStr=Inherit: Same as first input
  Sum11 : Sum  InputSameDT=on  SaturateOnIntegerOverflow=on  OutDataTypeStr=Inherit: Same as first input
  Sum13 : Sum  InputSameDT=on  SaturateOnIntegerOverflow=on  OutDataTypeStr=Inherit: Same as first input
  Trigonometric Function10 : Trigonometry
  Trigonometric Function11 : Trigonometry
  Trigonometric Function12 : Trigonometry  Operator=cos
  Trigonometric Function7 : Trigonometry  Operator=cos
  Trigonometric Function8 : Trigonometry
  Trigonometric Function9 : Trigonometry  Operator=cos
  abc : Outport
  wires:
  Trigonometric Function7/1 -> Product7/2
  Constant6/1 -> Sum10/1
  Sum7/1 -> Gain3/1
  Trigonometric Function11/1 -> Product11/2
  Constant5/1 -> Sum9/1
  Product10/1 -> Sum8/1
  Sum11/1 -> Trigonometric Function11/1
  Demux2/3 -> Trigonometric Function8/1, Trigonometric Function7/1
  Demux2/2 -> Product8/1  "q"
  Demux2/1 -> Product7/1  "d"
  Demux3/2 -> Product10/1  "q"
  Product7/1 -> Sum7/2
  Trigonometric Function9/1 -> Product9/2
  Mux/1 -> Demux4/1, Demux2/1, Demux3/1
  Trigonometric Function12/1 -> Product12/2
  Sum13/1 -> Trigonometric Function12/1
  Sum10/1 -> Trigonometric Function10/1
  Trigonometric Function8/1 -> Product8/2
  Gain5/1 -> Mux1/3
  Sum8/1 -> Gain4/1
  Demux3/3 -> Sum10/2, Sum9/2
  Sum9/1 -> Trigonometric Function9/1
  Demux3/1 -> Product9/1  "d"
  Constant7/1 -> Sum13/1
  Demux4/3 -> Sum13/2, Sum11/2
  Product11/1 -> Sum12/1
  Demux4/1 -> Product12/1  "d"
  Demux4/2 -> Product11/1  "q"
  Gain4/1 -> Mux1/2
  Product8/1 -> Sum7/1
  Product9/1 -> Sum8/2
  Gain3/1 -> Mux1/1
  Product12/1 -> Sum12/2
  Constant8/1 -> Sum11/1
  Sum12/1 -> Gain5/1
  Trigonometric Function10/1 -> Product10/2
  Mux1/1 -> abc/1
  theta_d/1 -> Mux/2
  dq/1 -> Mux/1

== system WECSim_Lib_PTOSim/Electric/Direct Drive Rotary Generator/Losses ==
  vel : Inport
  Gain : Gain  Gain=ptoSim.directRotaryGenerator.Bfric
  fricTorque : Outport
  wires:
  vel/1 -> Gain/1
  Gain/1 -> fricTorque/1

== system WECSim_Lib_PTOSim/Electric/Direct Drive Rotary Generator/Subsystem ==
  vsdq : Inport
  wd : Inport  Port=2
  Add : Sum  Inputs=+-+
  Add1 : Sum  Inputs=--+
  Demux2 : Demux  Outputs=2
      settings: DisplayOption=none
  Fcn : Fcn  Expr=( u(1) - ptoSim.directRotaryGenerator.lambda_fd ) / ptoSim.directRotaryGenerator.Ls
  Gain : Gain  Gain=1/ptoSim.directRotaryGenerator.Ls
  Gain1 : Gain  Gain=pi*ptoSim.directRotaryGenerator.radius/ptoSim.directRotaryGenerator.tau_p*ptoSim.directRotaryGenerator.lambda_fd
  Gain2 : Gain  Gain=ptoSim.directRotaryGenerator.Rs
  Gain3 : Gain  Gain=ptoSim.directRotaryGenerator.Rs
  Integrator : Integrator  InitialCondition=ptoSim.directRotaryGenerator.lambda_sd_0
  Integrator1 : Integrator  InitialCondition=ptoSim.directRotaryGenerator.lambda_sq_0
  Mux : Mux  Inputs=2
  Product : Product  RndMeth=Zero
  Product1 : Product  RndMeth=Zero
  Fem : Outport
  isdq : Outport  Port=2
  wires:
  vsdq/1 -> Demux2/1  "vsdq"
  Gain1/1 -> Fem/1
  Mux/1 -> isdq/1  "isdq"
  Gain3/1 -> Add/2  "isd_Rs"
  Add/1 -> Integrator/1  "d_dt_lambda_sd"
  Integrator/1 -> Product1/2, Fcn/1  "lambda_sd"
  Add1/1 -> Integrator1/1  "d_dt_lambda_sq"
  Integrator1/1 -> Gain/1, Product/2  "lambda_sq"
  Demux2/1 -> Add/3  "vsd"
  Product1/1 -> Add1/1
  Demux2/2 -> Add1/3  "vsq"
  Gain2/1 -> Add1/2
  Fcn/1 -> Gain3/1, Mux/1  "isd"
  wd/1 -> Product1/1, Product/1
  Gain/1 -> Gain2/1, Mux/2, Gain1/1  "isq"
  Product/1 -> Add/1

== system WECSim_Lib_PTOSim/Electric/Direct Drive Rotary Generator/Subsystem1 ==
  Iabc : Inport
  Gain : Gain  Gain=-1
  Gain1 : Gain  Gain=ptoSim.directRotaryGenerator.Rload
  Product : Product
  Sum of Elements : Sum  Inputs=+
  Vabc : Outport
  elecPower : Outport  Port=2
  wires:
  Sum of Elements/1 -> Gain/1
  Iabc/1 -> Gain1/1, Product/2
  Product/1 -> Sum of Elements/1
  Gain/1 -> elecPower/1  "elecPower"
  Gain1/1 -> Vabc/1, Product/1

== system WECSim_Lib_PTOSim/Hydraulic/Check Valve/Subsystem ==
  DeltaP : Inport
  Add : Sum
  Add1 : Sum  Inputs=+-
  Add2 : Sum  Inputs=+-
  Add3 : Sum
  Add4 : Sum
  Constant : Constant
  Constant1 : Constant  Value=ptoSim.checkValve.Amax
  Constant2 : Constant  Value=ptoSim.checkValve.Amin
  Constant3 : Constant  Value=ptoSim.checkValve.pMax
  Constant4 : Constant  Value=ptoSim.checkValve.pMin
  Constant5 : Constant  Value=ptoSim.checkValve.Amin
  Gain : Gain  Gain=ptoSim.checkValve.k2
  Gain1 : Gain  Gain=0.5
  Gain2 : Gain  Gain=0.5
  Product : Product
  Trigonometric Function : Trigonometry  Operator=tanh
  Av : Outport
  wires:
  Gain1/1 -> Add2/2
  Add2/1 -> Gain/1
  Constant3/1 -> Add3/1
  Constant4/1 -> Add3/2
  Constant2/1 -> Add1/2
  Product/1 -> Add4/2
  Constant5/1 -> Add4/1
  Gain/1 -> Trigonometric Function/1
  DeltaP/1 -> Add2/1
  Constant/1 -> Add/2
  Add1/1 -> Gain2/1
  Gain2/1 -> Product/2
  Trigonometric Function/1 -> Add/1
  Add3/1 -> Gain1/1
  Add/1 -> Product/1
  Constant1/1 -> Add1/1
  Add4/1 -> Av/1

== system WECSim_Lib_PTOSim/Hydraulic/Compressible Fluid Piston/Subsystem ==
  Pos : Inport
  Vel : Inport  Port=2
  QB : Inport  Port=3
  Add : Sum  Inputs=-+
  Add1 : Sum  Inputs=+-+
  Constant : Constant  Value=ptoSim.hydPistonCompressible.Ap_B
  Constant1 : Constant  Value=ptoSim.hydPistonCompressible.pistonStroke
  Constant2 : Constant  Value=ptoSim.hydPistonCompressible.Ap_B
  Constant3 : Constant  Value=ptoSim.hydPistonCompressible.bulkModulus
  Constant4 : Constant  Value=ptoSim.hydPistonCompressible.xi_piston
  Divide : Product  Inputs=/*
  Product : Product
  Product1 : Product
  Product2 : Product
  Saturation : Saturate  UpperLimit=inf  LowerLimit=1e-10
  dPB_dt : Outport
  wires:
  Saturation/1 -> Divide/1
  Vel/1 -> Product/1
  Constant/1 -> Product/2
  Product/1 -> Add/1
  QB/1 -> Add/2
  Add/1 -> Product1/2
  Pos/1 -> Add1/1
  Add1/1 -> Product2/1
  Constant2/1 -> Product2/2
  Product2/1 -> Saturation/1
  Constant3/1 -> Divide/2
  Divide/1 -> Product1/1
  Product1/1 -> dPB_dt/1
  Constant1/1 -> Add1/3
  Constant4/1 -> Add1/2
